simulink model "FSI05"  (R2024b)
settings: Solver=FixedStepAuto  StartTime=0.0  StopTime=4  FixedStep=0.0001  RelTol=1e-3
values from neighbouring files (symbols this model uses):
  cphi = 0.1    [FSI05WS.m]    (also in FSI06WS.m; FSI07WS.m)
  I0 = 0    [FSI03WS.m]    (also in FSI05WS.m = 0.0001; FSI06WS.m = 0.0001; FSI07WS.m = 0.0001)
  L = 0.02    [FSI03WS.m]    (also in FSI05WS.m = 0.05; FSI06WS.m = 0.05; FSI07WS.m = 0.05; FSI10WS.m = 0.3)
  M = 0    [FSI05WS.m]    (also in FSI06WS.m = 0.2; FSI07WS.m = 0.04; FSI10WS.m = 3)
  R = 5    [FSI03WS.m]    (also in FSI05WS.m = 0; FSI06WS.m = 20; FSI07WS.m = 20)
  step_t = 2    [FSI05WS.m]    (also in FSI06WS.m = 1; FSI07WS.m = 0.5)
  U = 10    [FSI03WS.m]    (also in FSI05WS.m = 24; FSI06WS.m = 24)
settings Model: Creator=fmiro  LastModifiedBy=fmiro

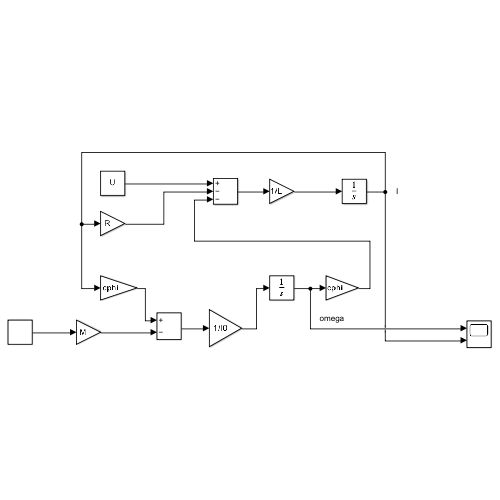
[thumbnail: Simulink's stored preview of the top-level diagram]
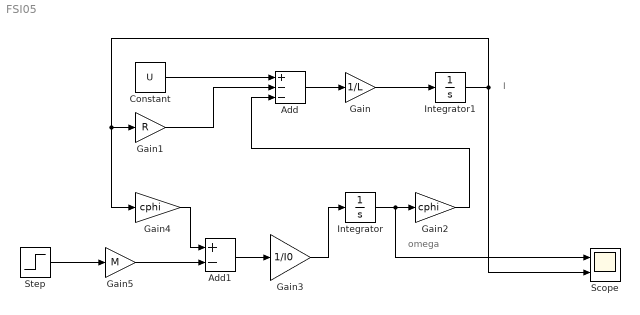
== system FSI05 ==
  note: omega
  note: I
  Add : Sum  Inputs=+--
  Add1 : Sum  Inputs=+-
  Constant : Constant  Value=U
  Gain : Gain  Gain=1/L
  Gain1 : Gain  Gain=R
  Gain2 : Gain  Gain=cphi
  Gain3 : Gain  Gain=1/I0
  Gain4 : Gain  Gain=cphi
  Gain5 : Gain  Gain=M
  Integrator : Integrator
  Integrator1 : Integrator
  Scope : Scope  NumInputPorts=2
  Step : Step  Time=step_t  SampleTime=0
  wires:
  Constant/1 -> Add/1
  Gain1/1 -> Add/2
  Integrator/1 -> Scope/1, Gain2/1
  Add/1 -> Gain/1
  Gain2/1 -> Add/3
  Gain/1 -> Integrator1/1
  Integrator1/1 -> Scope/2, Gain4/1, Gain1/1
  Add1/1 -> Gain3/1
  Gain4/1 -> Add1/1
  Gain5/1 -> Add1/2
  Gain3/1 -> Integrator/1
  Step/1 -> Gain5/1
